simulink model "ACC5v_F_traingdx_15_15_15_controller_ep_50_Nor_20250702"  (R2021a)
settings: Solver=VariableStepAuto  StartTime=0.0  StopTime=10.0  RelTol=1e-3
libraries: neural x50
(part 2 of 2)

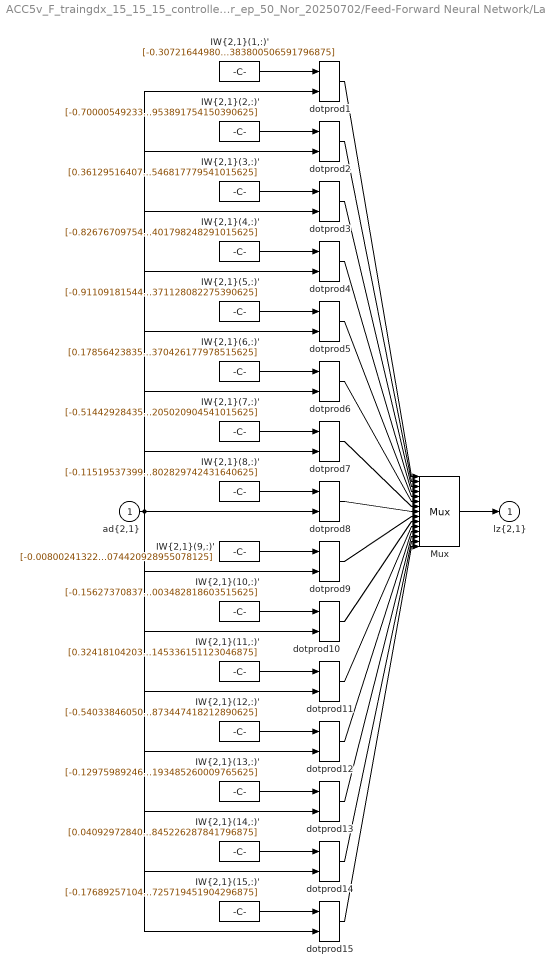
== system ACC5v_F_traingdx_15_15_15_controller_ep_50_Nor_20250702/Feed-Forward Neural Network/Layer 2/LW{2,1} ==
  "ad{2,1}" : Inport  PortDimensions=15
      mask Display: e = 0.06;c1 = [120 230 180]/255;c2 = ([120 230 180]+0)/(256+128);c3 = ([120 230 180]+128)/(256+128);patch([0 1 1 0],[0 0 1 1],c1);patch([0 1 1 1-e 1-e 0+e],[0 0 1 1-e 0+e 0+e],c2);patch([0 0 1 1-e 0+e 0+e],[0 1 1 1-e 1-e 0+e],c3);plot([0 1 1 0 0],[0 0 1 1 0]);
  "IW{2,1}(1,:)'" : Constant  Value=[-0.307216449809228520084758429220528341829776763916015625;-0.9608441683962196666612953777075745165348052978515625;0.57856846145458862284982615165063180029392242431640625;-0.1860903257221864226522711760480888187885284423828125;0.7014253456693582133851805338053964078426361083984375;-0.54431412858791627940036050858907401561737060546875;0.5380581706717924017624454791075550019741058349609375;-0.9009348419158775822523921306128613650798797607421875;-0.7521354448038597428904949993011541664600372314453125;0.241917287870616615208518851432017982006072998046875;-0.7321374980240575869316899115801788866519927978515625;-0.6457849324217816988635831876308657228946685791015625;-0.643766092226467190329231016221456229686737060546875;-0.63161180496894697711240951321087777614593505859375;-0.095583894851617390298059717679279856383800506591796875]
      mask Display: e = 0.06;c1 = [120 150 230]/255;c2 = ([120 150 230]+0)/383;c3 = ([120 150 230]+128)/383;patch([0 1 1 0],[0 0 1 1],c1);patch([0 1 1 1-e 1-e 0+e],[0 0 1 1-e 0+e 0+e],c2);patch([0 0 1 1-e 0+e 0+e],[0 1 1 1-e 1-e 0+e],c3);plot([0 1 1 0 0],[0 0 1 1 0]);disp('weights');
  "IW{2,1}(10,:)'" : Constant  Value=[-0.1562737083758140854694573818051139824092388153076171875;0.538185902284831652053753714426420629024505615234375;1.0855152157811878144144657198921777307987213134765625;0.3573046096003764660054002888500690460205078125;0.73087720618158780183648559614084661006927490234375;-0.75784510969678298142326866582152433693408966064453125;-0.581189831958130564970588238793425261974334716796875;-0.4362662882391401542037101535242982208728790283203125;-0.588048968935513283184945976245217025279998779296875;0.968796624481943258189176049199886620044708251953125;0.6844132248386689543195871010539121925830841064453125;-0.364644190893188169244609753150143660604953765869140625;-0.01128810561224428965498844945614109747111797332763671875;-0.1165558858711521761364338090061210095882415771484375;0.5670219131222167252559529515565373003482818603515625]
      mask Display: e = 0.06;c1 = [120 150 230]/255;c2 = ([120 150 230]+0)/383;c3 = ([120 150 230]+128)/383;patch([0 1 1 0],[0 0 1 1],c1);patch([0 1 1 1-e 1-e 0+e],[0 0 1 1-e 0+e 0+e],c2);patch([0 0 1 1-e 0+e 0+e],[0 1 1 1-e 1-e 0+e],c3);plot([0 1 1 0 0],[0 0 1 1 0]);disp('weights');
  "IW{2,1}(11,:)'" : Constant  Value=[0.32418104203954356545835935321520082652568817138671875;-0.2069110601716603603517086185092921368777751922607421875;-0.07278199672912992468365445120070944540202617645263671875;-0.0096459618206787833827320355339907109737396240234375;0.2251329070069356397265636360316420905292034149169921875;0.1775307195497353440760690546085243113338947296142578125;0.1045826830775500315695580866304226219654083251953125;0.07719335609068078696282100281678140163421630859375;0.8958662425863372913426019295002333819866180419921875;0.7178776333677323595594543803599663078784942626953125;0.118065089977390069719831444672308862209320068359375;-0.230235005726832919759061724107596091926097869873046875;0.773460496912098616206776569015346467494964599609375;-0.97343359906549498106187456869520246982574462890625;0.1281059631437126977715479370090179145336151123046875]
      mask Display: e = 0.06;c1 = [120 150 230]/255;c2 = ([120 150 230]+0)/383;c3 = ([120 150 230]+128)/383;patch([0 1 1 0],[0 0 1 1],c1);patch([0 1 1 1-e 1-e 0+e],[0 0 1 1-e 0+e 0+e],c2);patch([0 0 1 1-e 0+e 0+e],[0 1 1 1-e 1-e 0+e],c3);plot([0 1 1 0 0],[0 0 1 1 0]);disp('weights');
  "IW{2,1}(12,:)'" : Constant  Value=[-0.54033846050153322426723434546147473156452178955078125;0.6164070674625785617450901554548181593418121337890625;0.469287110755986447419019214066793210804462432861328125;-0.6205791879648396847102276296936906874179840087890625;0.9799003580082541464690848442842252552509307861328125;0.110491742785650881586434479686431586742401123046875;0.25976677012884241690926501178182661533355712890625;0.390326078888663996480090645491145551204681396484375;-0.835857585804548275376646415679715573787689208984375;0.571117978530061076725132807041518390178680419921875;0.70819989854688625285916714346967637538909912109375;-0.2384282960007702290017306268055108375847339630126953125;-0.93545641092668618821193149415194056928157806396484375;0.794382701947144109766441033571027219295501708984375;-0.89437668890706911728472050526761449873447418212890625]
      mask Display: e = 0.06;c1 = [120 150 230]/255;c2 = ([120 150 230]+0)/383;c3 = ([120 150 230]+128)/383;patch([0 1 1 0],[0 0 1 1],c1);patch([0 1 1 1-e 1-e 0+e],[0 0 1 1-e 0+e 0+e],c2);patch([0 0 1 1-e 0+e 0+e],[0 1 1 1-e 1-e 0+e],c3);plot([0 1 1 0 0],[0 0 1 1 0]);disp('weights');
  "IW{2,1}(13,:)'" : Constant  Value=[-0.129759892462285808534261377644725143909454345703125;0.5091219139535063664681047157500870525836944580078125;-0.27503912869079172320851967015187256038188934326171875;-0.0099883500195583341252358877682127058506011962890625;0.055360058729363080531893359648165642283856868743896484375;0.14065699681347521021734792157076299190521240234375;-0.9360179684748661799176261411048471927642822265625;-0.0017679730348210132007125139352865517139434814453125;-0.7885811468365571119676360467565245926380157470703125;0.0267548371751498148540804322692565619945526123046875;-0.3042416113454777804037121313740499317646026611328125;0.274309830095190998466847531744861043989658355712890625;0.2748859603346549551616817552712745964527130126953125;-0.606683617264736074758957329322583973407745361328125;-0.95023231125094176352519070860580541193485260009765625]
      mask Display: e = 0.06;c1 = [120 150 230]/255;c2 = ([120 150 230]+0)/383;c3 = ([120 150 230]+128)/383;patch([0 1 1 0],[0 0 1 1],c1);patch([0 1 1 1-e 1-e 0+e],[0 0 1 1-e 0+e 0+e],c2);patch([0 0 1 1-e 0+e 0+e],[0 1 1 1-e 1-e 0+e],c3);plot([0 1 1 0 0],[0 0 1 1 0]);disp('weights');
  "IW{2,1}(14,:)'" : Constant  Value=[0.040929728407948971768970380935570574365556240081787109375;-0.2457279271460333369692108362869475968182086944580078125;-0.9554839555694261132856581753003410995006561279296875;-0.7047835560466226834108738330542109906673431396484375;-0.040953311119333722645219353353240876458585262298583984375;0.59630529781441976577838204320869408547878265380859375;0.2294268382342810053131643144297413527965545654296875;0.071602111502226506445367704145610332489013671875;-0.7159177561920035959275310233351774513721466064453125;-0.644795078988269931841159632313065230846405029296875;-0.1079467038897943265141066149226389825344085693359375;0.489196875011608245387151328031904995441436767578125;0.3450077880449369249760138700366951525211334228515625;-0.8132589664898139947268873584107495844364166259765625;0.2482096087059904032656731942552141845226287841796875]
      mask Display: e = 0.06;c1 = [120 150 230]/255;c2 = ([120 150 230]+0)/383;c3 = ([120 150 230]+128)/383;patch([0 1 1 0],[0 0 1 1],c1);patch([0 1 1 1-e 1-e 0+e],[0 0 1 1-e 0+e 0+e],c2);patch([0 0 1 1-e 0+e 0+e],[0 1 1 1-e 1-e 0+e],c3);plot([0 1 1 0 0],[0 0 1 1 0]);disp('weights');
  "IW{2,1}(15,:)'" : Constant  Value=[-0.176892571045714153132877299867686815559864044189453125;-0.5680516185601103273938861093483865261077880859375;-0.62049157476371774588841390141169540584087371826171875;-0.890051706187623636878925026394426822662353515625;0.60269518787856046770912143983878195285797119140625;0.9646064183901206234850178589113056659698486328125;-0.2751770754538946928136056158109568059444427490234375;-0.10963366940791541281896570581011474132537841796875;-0.667079118247158486809667010675184428691864013671875;-0.2028210065283138074931912342435680329799652099609375;-0.891521031117740836435814344440586864948272705078125;-0.799556919609016869543438588152639567852020263671875;0.1230528149265766313380510155184310860931873321533203125;-0.3852662008241598545765782546368427574634552001953125;0.6183943368136002316504118425655178725719451904296875]
      mask Display: e = 0.06;c1 = [120 150 230]/255;c2 = ([120 150 230]+0)/383;c3 = ([120 150 230]+128)/383;patch([0 1 1 0],[0 0 1 1],c1);patch([0 1 1 1-e 1-e 0+e],[0 0 1 1-e 0+e 0+e],c2);patch([0 0 1 1-e 0+e 0+e],[0 1 1 1-e 1-e 0+e],c3);plot([0 1 1 0 0],[0 0 1 1 0]);disp('weights');
  "IW{2,1}(2,:)'" : Constant  Value=[-0.7000054923366338943679920703289099037647247314453125;-0.3382842395718579364682909726980142295360565185546875;0.8986078236995937995601479997276328504085540771484375;0.4974114364313828584585053249611519277095794677734375;0.1211190547097695802136740894638933241367340087890625;-0.003811417607220590753058786503970623016357421875;0.162892975750795532263737186440266668796539306640625;-0.0208600216453564968333012075163424015045166015625;-0.0192854130639636967003980316803790628910064697265625;0.147419529682396355241280616610310971736907958984375;-0.9382209025100969324029165363754145801067352294921875;0.325616123921948830144401654251851141452789306640625;-0.2807301730358393587749787911889143288135528564453125;0.19442270067570976976867314078845083713531494140625;-0.7966612127504897333807321047061122953891754150390625]
      mask Display: e = 0.06;c1 = [120 150 230]/255;c2 = ([120 150 230]+0)/383;c3 = ([120 150 230]+128)/383;patch([0 1 1 0],[0 0 1 1],c1);patch([0 1 1 1-e 1-e 0+e],[0 0 1 1-e 0+e 0+e],c2);patch([0 0 1 1-e 0+e 0+e],[0 1 1 1-e 1-e 0+e],c3);plot([0 1 1 0 0],[0 0 1 1 0]);disp('weights');
  "IW{2,1}(3,:)'" : Constant  Value=[0.361295164077490793541613811612478457391262054443359375;-0.1507570216686442698961201358542894013226032257080078125;-0.1630865612170136758063421211772947572171688079833984375;0.6511676315723111674316214703139849007129669189453125;0.8592177565757885826513984284247271716594696044921875;0.9602288960638192261143331052153371274471282958984375;0.856626124628375951175485170097090303897857666015625;-0.6149792078758504754176783535513095557689666748046875;0.7059963106816324884817959173233248293399810791015625;-0.8958442194282607573541099554859101772308349609375;0.8782834121390958870279064285568892955780029296875;-0.2121372392485184887878091331003815867006778717041015625;-0.7794180237122088072965198080055415630340576171875;-0.4001260198204221740780894833733327686786651611328125;0.87172374797359053477663337616831995546817779541015625]
      mask Display: e = 0.06;c1 = [120 150 230]/255;c2 = ([120 150 230]+0)/383;c3 = ([120 150 230]+128)/383;patch([0 1 1 0],[0 0 1 1],c1);patch([0 1 1 1-e 1-e 0+e],[0 0 1 1-e 0+e 0+e],c2);patch([0 0 1 1-e 0+e 0+e],[0 1 1 1-e 1-e 0+e],c3);plot([0 1 1 0 0],[0 0 1 1 0]);disp('weights');
  "IW{2,1}(4,:)'" : Constant  Value=[-0.8267670975429386448496416051057167351245880126953125;-0.45964561966120520697387519248877651989459991455078125;0.0258563792450836604785990857635624706745147705078125;0.579926059889061651375641304184682667255401611328125;0.3933344011104551452007171974400989711284637451171875;-0.0733611594085635532191957963732420466840267181396484375;0.1601807315168832790419628508971072733402252197265625;-0.753832504908109601871046834276057779788970947265625;0.7478548117234666836594669803162105381488800048828125;0.862402769216499276438980814418755471706390380859375;-0.3973878708272156057290658281999640166759490966796875;0.62012772528330295518372849983279593288898468017578125;-0.10838857987476979705121493680053390562534332275390625;-0.7317541343426352540291190962307155132293701171875;-0.413457841268517312105501559926779009401798248291015625]
      mask Display: e = 0.06;c1 = [120 150 230]/255;c2 = ([120 150 230]+0)/383;c3 = ([120 150 230]+128)/383;patch([0 1 1 0],[0 0 1 1],c1);patch([0 1 1 1-e 1-e 0+e],[0 0 1 1-e 0+e 0+e],c2);patch([0 0 1 1-e 0+e 0+e],[0 1 1 1-e 1-e 0+e],c3);plot([0 1 1 0 0],[0 0 1 1 0]);disp('weights');
  "IW{2,1}(5,:)'" : Constant  Value=[-0.9110918154435230231769082820392213761806488037109375;-0.6058924038090884867102658972726203501224517822265625;-0.122710034826088776327424056944437325000762939453125;-0.3629515092020156874497160970349796116352081298828125;0.165581930351680117752266596653498709201812744140625;0.6903563701080732695203323601162992417812347412109375;-0.96603412332547744512112330994568765163421630859375;-0.5890116581846402965538800344802439212799072265625;-0.45941133541460477118789640371687710285186767578125;0.457323363356542333946208600536920130252838134765625;-0.408932331049287167701322687207721173763275146484375;-0.763689603106578740465693044825457036495208740234375;-0.3283020506461509224749306667945347726345062255859375;-0.574796933282314181923311480204574763774871826171875;-0.4053063682241566656472286922507919371128082275390625]
      mask Display: e = 0.06;c1 = [120 150 230]/255;c2 = ([120 150 230]+0)/383;c3 = ([120 150 230]+128)/383;patch([0 1 1 0],[0 0 1 1],c1);patch([0 1 1 1-e 1-e 0+e],[0 0 1 1-e 0+e 0+e],c2);patch([0 0 1 1-e 0+e 0+e],[0 1 1 1-e 1-e 0+e],c3);plot([0 1 1 0 0],[0 0 1 1 0]);disp('weights');
  "IW{2,1}(6,:)'" : Constant  Value=[0.178564238353188187158337996152113191783428192138671875;0.64265492384980171802766335531487129628658294677734375;0.365648342633303979898329316711169667541980743408203125;0.0681282547414527872575717992731370031833648681640625;0.63079437011120986777967800662736408412456512451171875;0.264058630567132801569840694355661980807781219482421875;-0.7582808578028836787865429869270883500576019287109375;-0.7069701787702202810947937905439175665378570556640625;-0.5830772824973724510755346273072063922882080078125;0.4756833075951802936032208890537731349468231201171875;-0.3341274363276494074881384221953339874744415283203125;0.8071925900792422670093628767062909901142120361328125;-0.7930403375903603002683439626707695424556732177734375;0.789883350881628754081020815647207200527191162109375;-0.950883358085134577919461662531830370426177978515625]
      mask Display: e = 0.06;c1 = [120 150 230]/255;c2 = ([120 150 230]+0)/383;c3 = ([120 150 230]+128)/383;patch([0 1 1 0],[0 0 1 1],c1);patch([0 1 1 1-e 1-e 0+e],[0 0 1 1-e 0+e 0+e],c2);patch([0 0 1 1-e 0+e 0+e],[0 1 1 1-e 1-e 0+e],c3);plot([0 1 1 0 0],[0 0 1 1 0]);disp('weights');
  "IW{2,1}(7,:)'" : Constant  Value=[-0.5144292843580762220057067679590545594692230224609375;-0.140157181233467209580112466937862336635589599609375;0.537708504859229829975220127380453050136566162109375;-0.82009864245883790090374532155692577362060546875;0.7580278091943555285325828663189895451068878173828125;0.17197407165295164332974309218116104602813720703125;0.725421437399339286145050209597684442996978759765625;-0.621855651054772362584799338947050273418426513671875;0.1299591414764023067363041263888590037822723388671875;-0.8731909986143635560296161202131770551204681396484375;-0.065863625942295112025703929248265922069549560546875;0.0799641980758583059696320560760796070098876953125;-0.582106652013729242156614418490789830684661865234375;-0.8570943744259109653427231023670174181461334228515625;-0.40351205622447228194005219847895205020904541015625]
      mask Display: e = 0.06;c1 = [120 150 230]/255;c2 = ([120 150 230]+0)/383;c3 = ([120 150 230]+128)/383;patch([0 1 1 0],[0 0 1 1],c1);patch([0 1 1 1-e 1-e 0+e],[0 0 1 1-e 0+e 0+e],c2);patch([0 0 1 1-e 0+e 0+e],[0 1 1 1-e 1-e 0+e],c3);plot([0 1 1 0 0],[0 0 1 1 0]);disp('weights');
  "IW{2,1}(8,:)'" : Constant  Value=[-0.1151953739961133482694322083261795341968536376953125;0.7755419085127075451424616403528489172458648681640625;-0.665492909010556576987482912954874336719512939453125;-0.776588511613593102111963162315078079700469970703125;0.9778232321591782127967462656670249998569488525390625;-0.5065309480280502096860573146841488778591156005859375;-0.031406977575795025359184364788234233856201171875;-0.9146951781777132861606105507235042750835418701171875;0.2806236503255161718328736242256127297878265380859375;0.720881126076463818463935240288265049457550048828125;0.2963968129323142353115372316096909344196319580078125;0.413834838645525504574607111862860620021820068359375;0.8103071180089280733938039702479727566242218017578125;-0.5150268821265611141058116118074394762516021728515625;-0.90729747020363848974966458627022802829742431640625]
      mask Display: e = 0.06;c1 = [120 150 230]/255;c2 = ([120 150 230]+0)/383;c3 = ([120 150 230]+128)/383;patch([0 1 1 0],[0 0 1 1],c1);patch([0 1 1 1-e 1-e 0+e],[0 0 1 1-e 0+e 0+e],c2);patch([0 0 1 1-e 0+e 0+e],[0 1 1 1-e 1-e 0+e],c3);plot([0 1 1 0 0],[0 0 1 1 0]);disp('weights');
  "IW{2,1}(9,:)'" : Constant  Value=[-0.00800241322716114221458294508693143143318593502044677734375;-0.21793415984547681585326017739134840667247772216796875;0.36509938921376161591325626432080753147602081298828125;-0.727414902123402651312744637834839522838592529296875;-0.9989553102319643773654433971387334167957305908203125;0.059256121163638451887489821956478408537805080413818359375;0.6897113491525264095116654061712324619293212890625;0.270395833719764056013445951975882053375244140625;-0.16594209671422799345918974722735583782196044921875;0.8688102379224267313162499704048968851566314697265625;-0.9495436370139274107060600726981647312641143798828125;0.781641254626940007455004888470284640789031982421875;0.16424354700263166240148393626441247761249542236328125;-0.892491215582572383624437861726619303226470947265625;0.06124431775653001175374612330415402539074420928955078125]
      mask Display: e = 0.06;c1 = [120 150 230]/255;c2 = ([120 150 230]+0)/383;c3 = ([120 150 230]+128)/383;patch([0 1 1 0],[0 0 1 1],c1);patch([0 1 1 1-e 1-e 0+e],[0 0 1 1-e 0+e 0+e],c2);patch([0 0 1 1-e 0+e 0+e],[0 1 1 1-e 1-e 0+e],c3);plot([0 1 1 0 0],[0 0 1 1 0]);disp('weights');
  Mux : Mux  Inputs=15
      mask Display: e = 0.06;c1 = [120 150 230]/255;c2 = ([120 150 230]+0)/383;c3 = ([120 150 230]+128)/383;patch([0 1 1 0],[0 0 1 1],c1);patch([0 1 1 1-e 1-e 0+e],[0 0 1 1-e 0+e 0+e],c2);patch([0 0 1 1-e 0+e 0+e],[0 1 1 1-e 1-e 0+e],c3);plot([0 1 1 0 0],[0 0 1 1 0]);disp('Mux');
  dotprod{1..15} (15 alike) : neural/Weight Functions/dotprod
  "lz{2,1}" : Outport
      mask Display: e = 0.06;c1 = [120 230 180]/255;c2 = ([120 230 180]+0)/(256+128);c3 = ([120 230 180]+128)/(256+128);patch([0 1 1 0],[0 0 1 1],c1);patch([0 1 1 1-e 1-e 0+e],[0 0 1 1-e 0+e 0+e],c2);patch([0 0 1 1-e 0+e 0+e],[0 1 1 1-e 1-e 0+e],c3);plot([0 1 1 0 0],[0 0 1 1 0]);
  wires:
  "IW{2,1}(1,:)'"/1 -> dotprod1/1
  "ad{2,1}"/1 -> dotprod1/2, dotprod2/2, dotprod3/2, dotprod4/2, dotprod5/2, dotprod6/2, dotprod7/2, dotprod8/2, dotprod9/2, dotprod10/2, dotprod11/2, dotprod12/2, dotprod13/2, dotprod14/2, dotprod15/2
  dotprod1/1 -> Mux/1
  "IW{2,1}(2,:)'"/1 -> dotprod2/1
  dotprod2/1 -> Mux/2
  "IW{2,1}(3,:)'"/1 -> dotprod3/1
  dotprod3/1 -> Mux/3
  "IW{2,1}(4,:)'"/1 -> dotprod4/1
  dotprod4/1 -> Mux/4
  "IW{2,1}(5,:)'"/1 -> dotprod5/1
  dotprod5/1 -> Mux/5
  "IW{2,1}(6,:)'"/1 -> dotprod6/1
  dotprod6/1 -> Mux/6
  "IW{2,1}(7,:)'"/1 -> dotprod7/1
  dotprod7/1 -> Mux/7
  "IW{2,1}(8,:)'"/1 -> dotprod8/1
  dotprod8/1 -> Mux/8
  "IW{2,1}(9,:)'"/1 -> dotprod9/1
  dotprod9/1 -> Mux/9
  "IW{2,1}(10,:)'"/1 -> dotprod10/1
  dotprod10/1 -> Mux/10
  "IW{2,1}(11,:)'"/1 -> dotprod11/1
  dotprod11/1 -> Mux/11
  "IW{2,1}(12,:)'"/1 -> dotprod12/1
  dotprod12/1 -> Mux/12
  "IW{2,1}(13,:)'"/1 -> dotprod13/1
  dotprod13/1 -> Mux/13
  "IW{2,1}(14,:)'"/1 -> dotprod14/1
  dotprod14/1 -> Mux/14
  "IW{2,1}(15,:)'"/1 -> dotprod15/1
  dotprod15/1 -> Mux/15
  Mux/1 -> "lz{2,1}"/1

== system ACC5v_F_traingdx_15_15_15_controller_ep_50_Nor_20250702/Feed-Forward Neural Network/Layer 3/Delays 1 ==
  "p{3}" : Inport  PortDimensions=15
      mask Display: e = 0.06;c1 = [120 230 180]/255;c2 = ([120 230 180]+0)/(256+128);c3 = ([120 230 180]+128)/(256+128);patch([0 1 1 0],[0 0 1 1],c1);patch([0 1 1 1-e 1-e 0+e],[0 0 1 1-e 0+e 0+e],c2);patch([0 0 1 1-e 0+e 0+e],[0 1 1 1-e 1-e 0+e],c3);plot([0 1 1 0 0],[0 0 1 1 0]);
  mux : Mux  Inputs=1
      mask Display: e = 0.06;c1 = [120 150 230]/255;c2 = ([120 150 230]+0)/383;c3 = ([120 150 230]+128)/383;patch([0 1 1 0],[0 0 1 1],c1);patch([0 1 1 1-e 1-e 0+e],[0 0 1 1-e 0+e 0+e],c2);patch([0 0 1 1-e 0+e 0+e],[0 1 1 1-e 1-e 0+e],c3);plot([0 1 1 0 0],[0 0 1 1 0]);disp('Mux')
  "pd{3,2}" : Outport
      mask Display: e = 0.06;c1 = [120 230 180]/255;c2 = ([120 230 180]+0)/(256+128);c3 = ([120 230 180]+128)/(256+128);patch([0 1 1 0],[0 0 1 1],c1);patch([0 1 1 1-e 1-e 0+e],[0 0 1 1-e 0+e 0+e],c2);patch([0 0 1 1-e 0+e 0+e],[0 1 1 1-e 1-e 0+e],c3);plot([0 1 1 0 0],[0 0 1 1 0]);
  wires:
  "p{3}"/1 -> mux/1
  mux/1 -> "pd{3,2}"/1

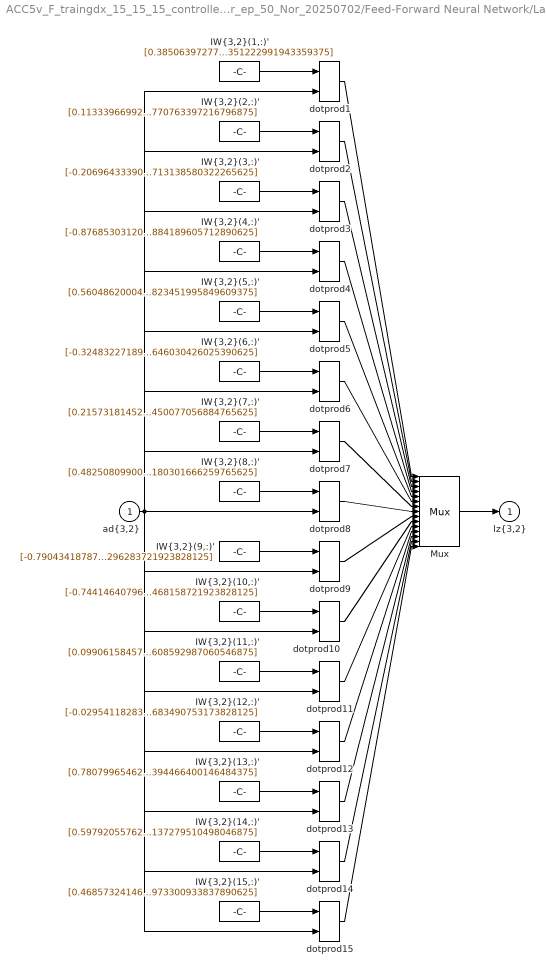
== system ACC5v_F_traingdx_15_15_15_controller_ep_50_Nor_20250702/Feed-Forward Neural Network/Layer 3/LW{3,2} ==
  "ad{3,2}" : Inport  PortDimensions=15
      mask Display: e = 0.06;c1 = [120 230 180]/255;c2 = ([120 230 180]+0)/(256+128);c3 = ([120 230 180]+128)/(256+128);patch([0 1 1 0],[0 0 1 1],c1);patch([0 1 1 1-e 1-e 0+e],[0 0 1 1-e 0+e 0+e],c2);patch([0 0 1 1-e 0+e 0+e],[0 1 1 1-e 1-e 0+e],c3);plot([0 1 1 0 0],[0 0 1 1 0]);
  "IW{3,2}(1,:)'" : Constant  Value=[0.3850639727730376105085952076478861272335052490234375;-0.897336227775257899708094555535353720188140869140625;0.19402719546265079220148663807776756584644317626953125;-0.61142673461330698803095629045856185257434844970703125;-0.7754320756879466980393544872640632092952728271484375;-0.391072049985144387651558872676105238497257232666015625;-0.81529532256159686909313677460886538028717041015625;-0.367142001707418064171406513196416199207305908203125;0.5269339366709495653395833869581110775470733642578125;-0.39869781404825410664471974087064154446125030517578125;-1.018482378139615729395472953910939395427703857421875;-0.154138719995460637957052085766918025910854339599609375;0.330846843751298635982749374306877143681049346923828125;0.48567415882336650856387905150768347084522247314453125;-0.45187343782479982845501353949657641351222991943359375]
      mask Display: e = 0.06;c1 = [120 150 230]/255;c2 = ([120 150 230]+0)/383;c3 = ([120 150 230]+128)/383;patch([0 1 1 0],[0 0 1 1],c1);patch([0 1 1 1-e 1-e 0+e],[0 0 1 1-e 0+e 0+e],c2);patch([0 0 1 1-e 0+e 0+e],[0 1 1 1-e 1-e 0+e],c3);plot([0 1 1 0 0],[0 0 1 1 0]);disp('weights');
  "IW{3,2}(10,:)'" : Constant  Value=[-0.74414640796159670088627535733394324779510498046875;-0.7650142956963341678289225455955602228641510009765625;0.1917891515194141138778149979771114885807037353515625;-0.411867332482743098154287508805282413959503173828125;0.3109960796070747601760331235709600150585174560546875;-0.8811934062834456682367090252228081226348876953125;-0.731393391372850754095225056516937911510467529296875;0.8276008215591357242146841599605977535247802734375;0.2434640897686779215103314299994963221251964569091796875;-0.1652074910540340113573876124064554460346698760986328125;0.5369835158974820554789175730547867715358734130859375;0.4054046139009506166672736071632243692874908447265625;-0.489226519023898465121646950137801468372344970703125;0.36527620530264215403803973458707332611083984375;0.74408080647514041050527566767414100468158721923828125]
      mask Display: e = 0.06;c1 = [120 150 230]/255;c2 = ([120 150 230]+0)/383;c3 = ([120 150 230]+128)/383;patch([0 1 1 0],[0 0 1 1],c1);patch([0 1 1 1-e 1-e 0+e],[0 0 1 1-e 0+e 0+e],c2);patch([0 0 1 1-e 0+e 0+e],[0 1 1 1-e 1-e 0+e],c3);plot([0 1 1 0 0],[0 0 1 1 0]);disp('weights');
  "IW{3,2}(11,:)'" : Constant  Value=[0.09906158457624598956403616512034204788506031036376953125;0.2814358459318511140878626974881626665592193603515625;0.50443284751643380214858325416571460664272308349609375;-0.5252539605888415508161415345966815948486328125;-0.780489898553896832567033925442956387996673583984375;-0.3683771233222679075680616733734495937824249267578125;-0.8028118145780045455950357791152782738208770751953125;0.4134304353938611509278189259930513799190521240234375;-0.69186988925645287462629084984655492007732391357421875;-0.313793336988434978795936558526591397821903228759765625;0.500873069898201350724775693379342555999755859375;-0.692819246761199547535170495393685996532440185546875;-0.9589284506836308619170949896215461194515228271484375;0.398339145900966473679005730446078814566135406494140625;0.2315624801974518476299635949544608592987060546875]
      mask Display: e = 0.06;c1 = [120 150 230]/255;c2 = ([120 150 230]+0)/383;c3 = ([120 150 230]+128)/383;patch([0 1 1 0],[0 0 1 1],c1);patch([0 1 1 1-e 1-e 0+e],[0 0 1 1-e 0+e 0+e],c2);patch([0 0 1 1-e 0+e 0+e],[0 1 1 1-e 1-e 0+e],c3);plot([0 1 1 0 0],[0 0 1 1 0]);disp('weights');
  "IW{3,2}(12,:)'" : Constant  Value=[-0.029541182830081336163630112423561513423919677734375;-0.342371570486394549703845768817700445652008056640625;-0.408333763348794509528971730105695314705371856689453125;0.022303420144101936128944174697608104906976222991943359375;0.86751969677066487207639511325396597385406494140625;-0.088846625074300078495070920325815677642822265625;-0.7159455031361432464365179839660413563251495361328125;0.1155779335097524285203007821110077202320098876953125;-1.014736771953200555884677669382654130458831787109375;0.0945794001316613008878420032488065771758556365966796875;0.102323495247317819423216178620350547134876251220703125;0.7672344390510021927553907516994513571262359619140625;0.3493785515360239291027255603694356977939605712890625;-0.176400270600250708152856304877786897122859954833984375;-0.2898526962423020325587685874779708683490753173828125]
      mask Display: e = 0.06;c1 = [120 150 230]/255;c2 = ([120 150 230]+0)/383;c3 = ([120 150 230]+128)/383;patch([0 1 1 0],[0 0 1 1],c1);patch([0 1 1 1-e 1-e 0+e],[0 0 1 1-e 0+e 0+e],c2);patch([0 0 1 1-e 0+e 0+e],[0 1 1 1-e 1-e 0+e],c3);plot([0 1 1 0 0],[0 0 1 1 0]);disp('weights');
  "IW{3,2}(13,:)'" : Constant  Value=[0.78079965462902201078776442955131642520427703857421875;0.3076240451915472906563309152261354029178619384765625;-0.6245383768847128092005505095585249364376068115234375;-0.7871989426698799974246867350302636623382568359375;-0.62507838715662700224129366688430309295654296875;0.90611545101317947370489491731859743595123291015625;-0.6634974030169444869642347839544527232646942138671875;-0.3731420201268174086095541497343219816684722900390625;-0.05358542844748682976163678404191159643232822418212890625;0.448933842983587627628594418638385832309722900390625;0.74305049298066006002727590384893119335174560546875;0.194708717061383318469580672172014601528644561767578125;0.71094163956368394696738732818630523979663848876953125;0.10679348235890574747575243463870720006525516510009765625;0.911985915592127494022633982240222394466400146484375]
      mask Display: e = 0.06;c1 = [120 150 230]/255;c2 = ([120 150 230]+0)/383;c3 = ([120 150 230]+128)/383;patch([0 1 1 0],[0 0 1 1],c1);patch([0 1 1 1-e 1-e 0+e],[0 0 1 1-e 0+e 0+e],c2);patch([0 0 1 1-e 0+e 0+e],[0 1 1 1-e 1-e 0+e],c3);plot([0 1 1 0 0],[0 0 1 1 0]);disp('weights');
  "IW{3,2}(14,:)'" : Constant  Value=[0.597920557625758686270955877262167632579803466796875;0.498262926207038159276407895958982408046722412109375;-0.8266669052089354874368609671364538371562957763671875;-0.189369160238817446639814079389907419681549072265625;-0.4676423221847223476999033664469607174396514892578125;-0.7493356377816400293312426583725027740001678466796875;-0.6075021554860893235883168017608113586902618408203125;-0.6675928741956986822714270601863972842693328857421875;0.516224862654837135522711832891218364238739013671875;-0.1513304327486186817708357921219430863857269287109375;-0.7881591665344693797834452198003418743610382080078125;0.3594677964209338494327994339982978999614715576171875;0.8652271440971281979415152818546630442142486572265625;-0.2184758355916509575678219334804452955722808837890625;-0.551657002033745680336096484097652137279510498046875]
      mask Display: e = 0.06;c1 = [120 150 230]/255;c2 = ([120 150 230]+0)/383;c3 = ([120 150 230]+128)/383;patch([0 1 1 0],[0 0 1 1],c1);patch([0 1 1 1-e 1-e 0+e],[0 0 1 1-e 0+e 0+e],c2);patch([0 0 1 1-e 0+e 0+e],[0 1 1 1-e 1-e 0+e],c3);plot([0 1 1 0 0],[0 0 1 1 0]);disp('weights');
  "IW{3,2}(15,:)'" : Constant  Value=[0.4685732414603336337677319534122943878173828125;0.1663714629097523545198100691777653992176055908203125;0.448167082555654017195223559610894881188869476318359375;-0.770036804482072678723625358543358743190765380859375;0.5956605204231941730341759466682560741901397705078125;-0.41370408483396692300715358214802108705043792724609375;-0.36504044970112925483363142120651900768280029296875;0.244994518559790375178408794454298913478851318359375;1.13856593845504061590645505930297076702117919921875;-0.1979153211205989248977488159653148613870143890380859375;0.50871216642184580170038543656119145452976226806640625;-0.8550857550000630080688779344200156629085540771484375;-0.41704282506552192710813642406719736754894256591796875;0.77489192681789587080487535786232911050319671630859375;0.2241917021035507995296853778199874795973300933837890625]
      mask Display: e = 0.06;c1 = [120 150 230]/255;c2 = ([120 150 230]+0)/383;c3 = ([120 150 230]+128)/383;patch([0 1 1 0],[0 0 1 1],c1);patch([0 1 1 1-e 1-e 0+e],[0 0 1 1-e 0+e 0+e],c2);patch([0 0 1 1-e 0+e 0+e],[0 1 1 1-e 1-e 0+e],c3);plot([0 1 1 0 0],[0 0 1 1 0]);disp('weights');
  "IW{3,2}(2,:)'" : Constant  Value=[0.1133396699280251329611246546846814453601837158203125;-0.854229401802047760838831891305744647979736328125;-0.530346170504191416483763532596640288829803466796875;-0.2234567379043965740237354111741296947002410888671875;0.5688557814878254514923128226655535399913787841796875;0.5379165281177382684774102017399854958057403564453125;-0.9843594128613302185470956828794442117214202880859375;-0.564873381154358700229067835607565939426422119140625;-0.6591359538862333611319854753674007952213287353515625;0.3710714174950744403957969552720896899700164794921875;-0.951131967899252028786349910660646855831146240234375;-0.5756735894901312544646998503594659268856048583984375;0.4972377435523942512674011595663614571094512939453125;0.589315770777506298117032201844267547130584716796875;0.6290795458013025420740405024844221770763397216796875]
      mask Display: e = 0.06;c1 = [120 150 230]/255;c2 = ([120 150 230]+0)/383;c3 = ([120 150 230]+128)/383;patch([0 1 1 0],[0 0 1 1],c1);patch([0 1 1 1-e 1-e 0+e],[0 0 1 1-e 0+e 0+e],c2);patch([0 0 1 1-e 0+e 0+e],[0 1 1 1-e 1-e 0+e],c3);plot([0 1 1 0 0],[0 0 1 1 0]);disp('weights');
  "IW{3,2}(3,:)'" : Constant  Value=[-0.2069643339018674144114129376248456537723541259765625;-0.8229450806505591575756852762424387037754058837890625;0.53920070863062752319905257536447606980800628662109375;0.103557063914454960951161410775966942310333251953125;-0.416859364186138225960576164652593433856964111328125;-0.2079865095642496886085837104474194347858428955078125;-0.1537812296716669635543439653702080249786376953125;-0.4979163079685278159303152278880588710308074951171875;-0.48545323060982636942384260692051611840724945068359375;-0.407123250544257853089646914668264798820018768310546875;-0.380667418343543229042325037880800664424896240234375;-0.8029625246237832580931126358336769044399261474609375;-0.7596259640258387069167156369076110422611236572265625;0.24238980483716687785999965853989124298095703125;0.63931516994974180168043176308856345713138580322265625]
      mask Display: e = 0.06;c1 = [120 150 230]/255;c2 = ([120 150 230]+0)/383;c3 = ([120 150 230]+128)/383;patch([0 1 1 0],[0 0 1 1],c1);patch([0 1 1 1-e 1-e 0+e],[0 0 1 1-e 0+e 0+e],c2);patch([0 0 1 1-e 0+e 0+e],[0 1 1 1-e 1-e 0+e],c3);plot([0 1 1 0 0],[0 0 1 1 0]);disp('weights');
  "IW{3,2}(4,:)'" : Constant  Value=[-0.87685303120929403153382963864714838564395904541015625;0.5967017282279047929449689036118797957897186279296875;0.8627194160058220262499162345193326473236083984375;-0.5420934959537999642265049260458908975124359130859375;0.207066877501773660696926526725292205810546875;-0.4541224117526188042148760359850712120532989501953125;0.3111463498758286760903501999564468860626220703125;0.785844810571953988898030729615129530429840087890625;-0.20749807684014598407884477637708187103271484375;0.0264997487508386551924299823213004856370389461517333984375;-0.384302501327633161398722450030618347227573394775390625;0.64714894785567711466001128428615629673004150390625;0.0500903295252175251306425707298330962657928466796875;-0.1549992955353705070820069522596895694732666015625;0.6715842861145802089595235884189605712890625]
      mask Display: e = 0.06;c1 = [120 150 230]/255;c2 = ([120 150 230]+0)/383;c3 = ([120 150 230]+128)/383;patch([0 1 1 0],[0 0 1 1],c1);patch([0 1 1 1-e 1-e 0+e],[0 0 1 1-e 0+e 0+e],c2);patch([0 0 1 1-e 0+e 0+e],[0 1 1 1-e 1-e 0+e],c3);plot([0 1 1 0 0],[0 0 1 1 0]);disp('weights');
  "IW{3,2}(5,:)'" : Constant  Value=[0.56048620004689453377721974902669899165630340576171875;0.8860162791414054606065064945141784846782684326171875;0.78094253853289996580855358843109570443630218505859375;0.283881240798374623324207277619279921054840087890625;0.928845334431802616137474615243263542652130126953125;-0.92553073185934398026120106806047260761260986328125;0.445845049384048675022995666950009763240814208984375;0.406446449112582097740187236922793090343475341796875;-0.848330311495987476888558376231230795383453369140625;0.66822202727918622588987318522413261234760284423828125;0.3381106442397034950175793710513971745967864990234375;-0.64998052523584082251772997551597654819488525390625;-0.3483327424735016553114519410883076488971710205078125;-0.416826080412973254407660306242178194224834442138671875;0.055008978273089946531282379282856709323823451995849609375]
      mask Display: e = 0.06;c1 = [120 150 230]/255;c2 = ([120 150 230]+0)/383;c3 = ([120 150 230]+128)/383;patch([0 1 1 0],[0 0 1 1],c1);patch([0 1 1 1-e 1-e 0+e],[0 0 1 1-e 0+e 0+e],c2);patch([0 0 1 1-e 0+e 0+e],[0 1 1 1-e 1-e 0+e],c3);plot([0 1 1 0 0],[0 0 1 1 0]);disp('weights');
  "IW{3,2}(6,:)'" : Constant  Value=[-0.3248322718959097965552018649759702384471893310546875;0.367431144816716237500031638774089515209197998046875;-0.9641435706090699664372323240968398749828338623046875;-0.0685508576739419506207440235812100581824779510498046875;-0.135030012059278003988538330304436385631561279296875;-0.25667101564819716497112267461488954722881317138671875;0.0624185871648774703857043277821503579616546630859375;0.1114758854387731812352058113901875913143157958984375;-0.371202656256162111247931534308008849620819091796875;0.1740005289267501087380196622689254581928253173828125;0.5534388730274457657287712208926677703857421875;-0.80570663287270127828065824360237456858158111572265625;-0.38071255244474933032705621371860615909099578857421875;0.065899979759383497945890439950744621455669403076171875;0.271322777722753816220802036696113646030426025390625]
      mask Display: e = 0.06;c1 = [120 150 230]/255;c2 = ([120 150 230]+0)/383;c3 = ([120 150 230]+128)/383;patch([0 1 1 0],[0 0 1 1],c1);patch([0 1 1 1-e 1-e 0+e],[0 0 1 1-e 0+e 0+e],c2);patch([0 0 1 1-e 0+e 0+e],[0 1 1 1-e 1-e 0+e],c3);plot([0 1 1 0 0],[0 0 1 1 0]);disp('weights');
  "IW{3,2}(7,:)'" : Constant  Value=[0.215731814525891518741218533250503242015838623046875;-0.735834088572874467359952177503146231174468994140625;-0.39159367112433518531844356402871198952198028564453125;-0.6963089497674668226778749158256687223911285400390625;0.3895043892358802661846084447461180388927459716796875;-0.14087108149629390396739836432971060276031494140625;-0.782364123453909154903840317274443805217742919921875;-0.631132664484693517437108312151394784450531005859375;-0.19522333460767615775921512977220118045806884765625;-0.3830062444946593647188137765624560415744781494140625;0.84119492143015983653953071552678011357784271240234375;0.3319744328222211660062157534412108361721038818359375;-0.20223849523360204472055556834675371646881103515625;-0.59818003821535226105510218985727988183498382568359375;0.8486349469385763288897805978194810450077056884765625]
      mask Display: e = 0.06;c1 = [120 150 230]/255;c2 = ([120 150 230]+0)/383;c3 = ([120 150 230]+128)/383;patch([0 1 1 0],[0 0 1 1],c1);patch([0 1 1 1-e 1-e 0+e],[0 0 1 1-e 0+e 0+e],c2);patch([0 0 1 1-e 0+e 0+e],[0 1 1 1-e 1-e 0+e],c3);plot([0 1 1 0 0],[0 0 1 1 0]);disp('weights');
  "IW{3,2}(8,:)'" : Constant  Value=[0.4825080990044359197099765879102051258087158203125;0.4454490793135317261430827784352004528045654296875;-0.307414008578099140489570118006668053567409515380859375;0.5512848094878701754595340389641933143138885498046875;0.5161985505789081773997395430342294275760650634765625;-0.2988187468236949140276692560291849076747894287109375;0.26353274705697771196355461142957210540771484375;-0.5759383149353585196195126627571880817413330078125;0.7177220905983203724787244937033392488956451416015625;-0.408585328293541605315652986973873339593410491943359375;-0.2050947620106299551512307743905694223940372467041015625;0.74423008184984895674318750025122426450252532958984375;-0.328633868763663350431869503154302947223186492919921875;-1.0185021339635780268650933066965080797672271728515625;-0.1120716899623792617290973794297315180301666259765625]
      mask Display: e = 0.06;c1 = [120 150 230]/255;c2 = ([120 150 230]+0)/383;c3 = ([120 150 230]+128)/383;patch([0 1 1 0],[0 0 1 1],c1);patch([0 1 1 1-e 1-e 0+e],[0 0 1 1-e 0+e 0+e],c2);patch([0 0 1 1-e 0+e 0+e],[0 1 1 1-e 1-e 0+e],c3);plot([0 1 1 0 0],[0 0 1 1 0]);disp('weights');
  "IW{3,2}(9,:)'" : Constant  Value=[-0.79043418787468266994977739159367047250270843505859375;-0.7792930387153027549373973670299164950847625732421875;0.315947066491624684037020642790594138205051422119140625;-0.7987873552751569850016721829888410866260528564453125;-0.1347153477057989601206600127625279128551483154296875;0.2197143385804321003007544277352280914783477783203125;-0.7470002693413941852185189418378286063671112060546875;-0.8453063837746463971001276149763725697994232177734375;-0.1973912308733933584914410630517522804439067840576171875;-0.1141747240383237105287861368196900002658367156982421875;-0.53763277823528998755620023075607605278491973876953125;0.0331164167025408406885844669886864721775054931640625;-0.63852447949041124530822344240732491016387939453125;0.497690179436046487015943284859531559050083160400390625;-0.9091136167777265075784498549182899296283721923828125]
      mask Display: e = 0.06;c1 = [120 150 230]/255;c2 = ([120 150 230]+0)/383;c3 = ([120 150 230]+128)/383;patch([0 1 1 0],[0 0 1 1],c1);patch([0 1 1 1-e 1-e 0+e],[0 0 1 1-e 0+e 0+e],c2);patch([0 0 1 1-e 0+e 0+e],[0 1 1 1-e 1-e 0+e],c3);plot([0 1 1 0 0],[0 0 1 1 0]);disp('weights');
  Mux : Mux  Inputs=15
      mask Display: e = 0.06;c1 = [120 150 230]/255;c2 = ([120 150 230]+0)/383;c3 = ([120 150 230]+128)/383;patch([0 1 1 0],[0 0 1 1],c1);patch([0 1 1 1-e 1-e 0+e],[0 0 1 1-e 0+e 0+e],c2);patch([0 0 1 1-e 0+e 0+e],[0 1 1 1-e 1-e 0+e],c3);plot([0 1 1 0 0],[0 0 1 1 0]);disp('Mux');
  dotprod{1..15} (15 alike) : neural/Weight Functions/dotprod
  "lz{3,2}" : Outport
      mask Display: e = 0.06;c1 = [120 230 180]/255;c2 = ([120 230 180]+0)/(256+128);c3 = ([120 230 180]+128)/(256+128);patch([0 1 1 0],[0 0 1 1],c1);patch([0 1 1 1-e 1-e 0+e],[0 0 1 1-e 0+e 0+e],c2);patch([0 0 1 1-e 0+e 0+e],[0 1 1 1-e 1-e 0+e],c3);plot([0 1 1 0 0],[0 0 1 1 0]);
  wires:
  "IW{3,2}(1,:)'"/1 -> dotprod1/1
  "ad{3,2}"/1 -> dotprod1/2, dotprod2/2, dotprod3/2, dotprod4/2, dotprod5/2, dotprod6/2, dotprod7/2, dotprod8/2, dotprod9/2, dotprod10/2, dotprod11/2, dotprod12/2, dotprod13/2, dotprod14/2, dotprod15/2
  dotprod1/1 -> Mux/1
  "IW{3,2}(2,:)'"/1 -> dotprod2/1
  dotprod2/1 -> Mux/2
  "IW{3,2}(3,:)'"/1 -> dotprod3/1
  dotprod3/1 -> Mux/3
  "IW{3,2}(4,:)'"/1 -> dotprod4/1
  dotprod4/1 -> Mux/4
  "IW{3,2}(5,:)'"/1 -> dotprod5/1
  dotprod5/1 -> Mux/5
  "IW{3,2}(6,:)'"/1 -> dotprod6/1
  dotprod6/1 -> Mux/6
  "IW{3,2}(7,:)'"/1 -> dotprod7/1
  dotprod7/1 -> Mux/7
  "IW{3,2}(8,:)'"/1 -> dotprod8/1
  dotprod8/1 -> Mux/8
  "IW{3,2}(9,:)'"/1 -> dotprod9/1
  dotprod9/1 -> Mux/9
  "IW{3,2}(10,:)'"/1 -> dotprod10/1
  dotprod10/1 -> Mux/10
  "IW{3,2}(11,:)'"/1 -> dotprod11/1
  dotprod11/1 -> Mux/11
  "IW{3,2}(12,:)'"/1 -> dotprod12/1
  dotprod12/1 -> Mux/12
  "IW{3,2}(13,:)'"/1 -> dotprod13/1
  dotprod13/1 -> Mux/13
  "IW{3,2}(14,:)'"/1 -> dotprod14/1
  dotprod14/1 -> Mux/14
  "IW{3,2}(15,:)'"/1 -> dotprod15/1
  dotprod15/1 -> Mux/15
  Mux/1 -> "lz{3,2}"/1

== system ACC5v_F_traingdx_15_15_15_controller_ep_50_Nor_20250702/Feed-Forward Neural Network/Layer 4/Delays 1 ==
  "p{4}" : Inport  PortDimensions=15
      mask Display: e = 0.06;c1 = [120 230 180]/255;c2 = ([120 230 180]+0)/(256+128);c3 = ([120 230 180]+128)/(256+128);patch([0 1 1 0],[0 0 1 1],c1);patch([0 1 1 1-e 1-e 0+e],[0 0 1 1-e 0+e 0+e],c2);patch([0 0 1 1-e 0+e 0+e],[0 1 1 1-e 1-e 0+e],c3);plot([0 1 1 0 0],[0 0 1 1 0]);
  mux : Mux  Inputs=1
      mask Display: e = 0.06;c1 = [120 150 230]/255;c2 = ([120 150 230]+0)/383;c3 = ([120 150 230]+128)/383;patch([0 1 1 0],[0 0 1 1],c1);patch([0 1 1 1-e 1-e 0+e],[0 0 1 1-e 0+e 0+e],c2);patch([0 0 1 1-e 0+e 0+e],[0 1 1 1-e 1-e 0+e],c3);plot([0 1 1 0 0],[0 0 1 1 0]);disp('Mux')
  "pd{4,3}" : Outport
      mask Display: e = 0.06;c1 = [120 230 180]/255;c2 = ([120 230 180]+0)/(256+128);c3 = ([120 230 180]+128)/(256+128);patch([0 1 1 0],[0 0 1 1],c1);patch([0 1 1 1-e 1-e 0+e],[0 0 1 1-e 0+e 0+e],c2);patch([0 0 1 1-e 0+e 0+e],[0 1 1 1-e 1-e 0+e],c3);plot([0 1 1 0 0],[0 0 1 1 0]);
  wires:
  "p{4}"/1 -> mux/1
  mux/1 -> "pd{4,3}"/1

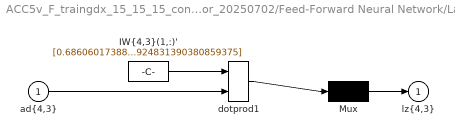
== system ACC5v_F_traingdx_15_15_15_controller_ep_50_Nor_20250702/Feed-Forward Neural Network/Layer 4/LW{4,3} ==
  "ad{4,3}" : Inport  PortDimensions=15
      mask Display: e = 0.06;c1 = [120 230 180]/255;c2 = ([120 230 180]+0)/(256+128);c3 = ([120 230 180]+128)/(256+128);patch([0 1 1 0],[0 0 1 1],c1);patch([0 1 1 1-e 1-e 0+e],[0 0 1 1-e 0+e 0+e],c2);patch([0 0 1 1-e 0+e 0+e],[0 1 1 1-e 1-e 0+e],c3);plot([0 1 1 0 0],[0 0 1 1 0]);
  "IW{4,3}(1,:)'" : Constant  Value=[0.6860601738812002192702266256674192845821380615234375;-0.2528723847147100745047509917640127241611480712890625;-0.83389528366286780336480433106771670281887054443359375;0.1396389090504018548610787320285453461110591888427734375;-0.67683142401064688709055872095632366836071014404296875;-0.0788416632700579267378770964569412171840667724609375;0.4317428577336575035161558844265528023242950439453125;-0.089850229650046242735328405615291558206081390380859375;0.27344387944233072840205522879841737449169158935546875;-0.380693910429242776682912108299206010997295379638671875;0.0730213687640452746574482034702668897807598114013671875;-0.05613117974812775745618864675634540617465972900390625;0.69765670549664504651588003980577923357486724853515625;0.6011173125576221298871359977056272327899932861328125;0.46817994213764535516020259819924831390380859375]
      mask Display: e = 0.06;c1 = [120 150 230]/255;c2 = ([120 150 230]+0)/383;c3 = ([120 150 230]+128)/383;patch([0 1 1 0],[0 0 1 1],c1);patch([0 1 1 1-e 1-e 0+e],[0 0 1 1-e 0+e 0+e],c2);patch([0 0 1 1-e 0+e 0+e],[0 1 1 1-e 1-e 0+e],c3);plot([0 1 1 0 0],[0 0 1 1 0]);disp('weights');
  Mux : Mux  Inputs=1
      mask Display: e = 0.06;c1 = [120 150 230]/255;c2 = ([120 150 230]+0)/383;c3 = ([120 150 230]+128)/383;patch([0 1 1 0],[0 0 1 1],c1);patch([0 1 1 1-e 1-e 0+e],[0 0 1 1-e 0+e 0+e],c2);patch([0 0 1 1-e 0+e 0+e],[0 1 1 1-e 1-e 0+e],c3);plot([0 1 1 0 0],[0 0 1 1 0]);disp('Mux');
  dotprod1 : neural/Weight Functions/dotprod
  "lz{4,3}" : Outport
      mask Display: e = 0.06;c1 = [120 230 180]/255;c2 = ([120 230 180]+0)/(256+128);c3 = ([120 230 180]+128)/(256+128);patch([0 1 1 0],[0 0 1 1],c1);patch([0 1 1 1-e 1-e 0+e],[0 0 1 1-e 0+e 0+e],c2);patch([0 0 1 1-e 0+e 0+e],[0 1 1 1-e 1-e 0+e],c3);plot([0 1 1 0 0],[0 0 1 1 0]);
  wires:
  "IW{4,3}(1,:)'"/1 -> dotprod1/1
  "ad{4,3}"/1 -> dotprod1/2
  dotprod1/1 -> Mux/1
  Mux/1 -> "lz{4,3}"/1
